simulink model "motor_plant"  (R2026a)
settings: Solver=ode4  StopTime=3  FixedStep=P_Ts/10
undefined symbols (not defined in the file or in its folder): P_Ts, PL_dz, PL_K, PL_Nrev, PL_tau, PL_td
settings Model: Creator=church  LastModifiedBy=church

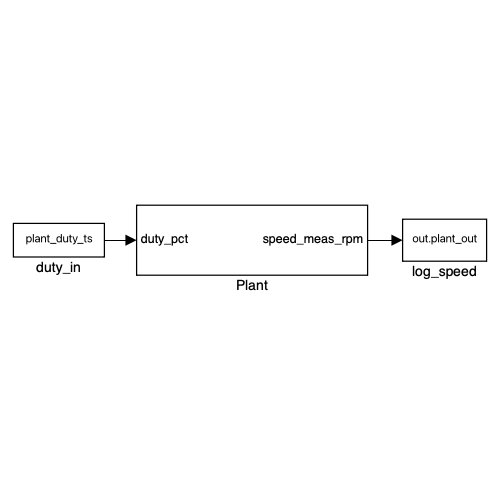
[thumbnail: Simulink's stored preview of the top-level diagram]
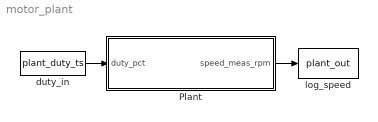
== system motor_plant ==
  Plant : Subsystem
  duty_in : FromWorkspace  VariableName=plant_duty_ts  SampleTime=P_Ts  Interpolate=off  OutputAfterFinalValue=Holding final value
  log_speed : ToWorkspace  VariableName=plant_out  SaveFormat=Timeseries  SampleTime=-1
  wires:
  Plant/1(speed_meas_rpm) -> log_speed/1
  duty_in/1 -> Plant/1(duty_pct)

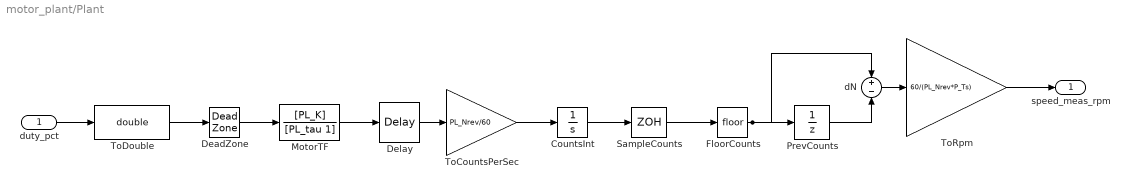
== system motor_plant/Plant ==
  duty_pct : Inport
  CountsInt : Integrator
  DeadZone : DeadZone  LowerValue=-PL_dz  UpperValue=PL_dz
  Delay : TransportDelay  DelayTime=PL_td
  FloorCounts : Rounding
  MotorTF : TransferFcn  Numerator=[PL_K]  Denominator=[PL_tau 1]
  PrevCounts : UnitDelay  SampleTime=P_Ts
  SampleCounts : ZeroOrderHold  SampleTime=P_Ts
  ToCountsPerSec : Gain  Gain=PL_Nrev/60
  ToDouble : DataTypeConversion  OutDataTypeStr=double  SaturateOnIntegerOverflow=off  RndMeth=Floor
  ToRpm : Gain  Gain=60/(PL_Nrev*P_Ts)
  dN : Sum  Inputs=+-
  speed_meas_rpm : Outport
  wires:
  ToRpm/1 -> speed_meas_rpm/1
  dN/1 -> ToRpm/1
  SampleCounts/1 -> FloorCounts/1
  ToDouble/1 -> DeadZone/1
  PrevCounts/1 -> dN/2
  DeadZone/1 -> MotorTF/1
  ToCountsPerSec/1 -> CountsInt/1
  Delay/1 -> ToCountsPerSec/1
  duty_pct/1 -> ToDouble/1
  MotorTF/1 -> Delay/1
  FloorCounts/1 -> PrevCounts/1, dN/1
  CountsInt/1 -> SampleCounts/1
